simulink model "modelClampedBeam"  (R2024b)
settings: Solver=ode4  StartTime=0.0  StopTime=inf  FixedStep=settings.samplingTime_s  MaxStep=1e-2  RelTol=1e-5
PostLoadFcn:
  | , if any(exist('dsrtsu_mdlpostloadfcn', 'file') == [2, 3, 6]), try dsrtsu_mdlpostloadfcn('Execute', bdroot); catch fprintf('Error in PostLoadFcn (dsrtsu_mdlpostloadfcn) for model "%s":\n %s\n', bdroot, lasterr); end, end,
  | , if any(exist('dsrtsu_mdlpostloadfcn', 'file') ~= 0), dsrtsu_mdlpostloadfcn('Execute', bdroot); end,
undefined symbols (not defined in the file or in its folder): virtualBeam
Description:
  | Standard RTI1202 template.
  | Supported MATLAB version:  R2019b.
settings Model: Tag=RTI1202  DSRTSU_INTERNAL_RTI_VER=490  DSRTSU_INTERNAL_RTI_TYPE=rti1202  RTICANMMDATA=struct('GeneralSetupData',struct('modelroot','C:\UNI\Master\04_MA\05_Experiments','generalsettings',struct('filesettings',struct('destfolder',struct('Name','RTICANMM_FILES','Check',1),'buildfolder',struct('Name','.','Check',1),'AbsDestfolder',struct('Name','C:\UNI\Master\04_MA\05_Experiments\RTICANMM_FILES'),'AbsBuildfolder',struct('Name','C:\UNI\Master\04_MA\05_Experiments'))),'options',struct('addpaths',1,'rmpaths',1,'addtrcexclusion',true,'cannavigator',struct('checkmonitoring',0),'show_usrtrc',0,'use_usrtrc',0),'advanced',struct('options',ones(1,100)),'MPSetup',{{}},'RTI',struct('Type','RTI1202','Ver','7.13','Date','02-Nov-2019'),'modelname','PLL_autoStep_r2019b_rti','block','PLL_autoStep_r2019b_rti'))  DSRTSU_INTERNAL_RTIFPGA=80  Creator=patri  LastModifiedBy=phippold
settings SolverCC: AlgebraicLoopSolver=TrustRegion
settings DataIOCC: ReturnWorkspaceOutputs=off
settings OptimizationCC: BlockReduction=off  OptimizeBlockIOStorage=off  BufferReuse=off  GlobalBufferReuse=off  ExpressionFolding=off  LocalBlockOutputs=off
settings DebuggingCC: UnconnectedInputMsg=warning  UnconnectedOutputMsg=warning  UnconnectedLineMsg=warning  ArithmeticOperatorsInVariantConditions=warning
settings HardwareCC: TargetIntDivRoundTo=Zero  TargetEndianess=BigEndian  TargetHWDeviceType=Custom Processor->Custom
settings ModelReferenceCC: EnableRefExpFcnMdlSchedulingChecks=on
settings SFSimCC: SimUseLocalCustomCode=off  CustomCodeUndefinedFunction=UseInterfaceOnly
settings RTWCC: RTWUseLocalCustomCode=off  GPUComputeCapability=3.5  DLArmComputeVersion=19.05
settings CodeAppCC: StateflowObjectComments=on
settings ConfigComp: CovMetricSettings=dswe
settings SimscapeCC: SimscapeNormalizeSystem=off

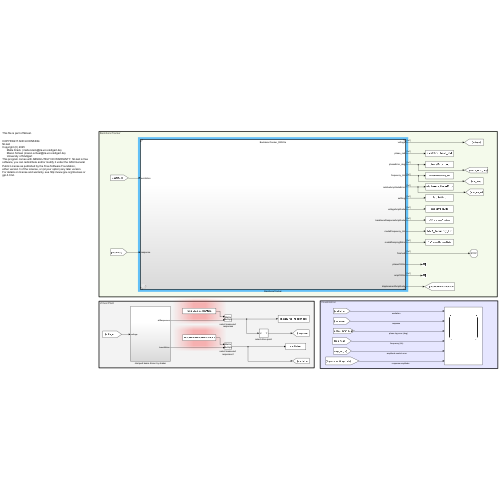
[thumbnail: Simulink's stored preview of the top-level diagram]
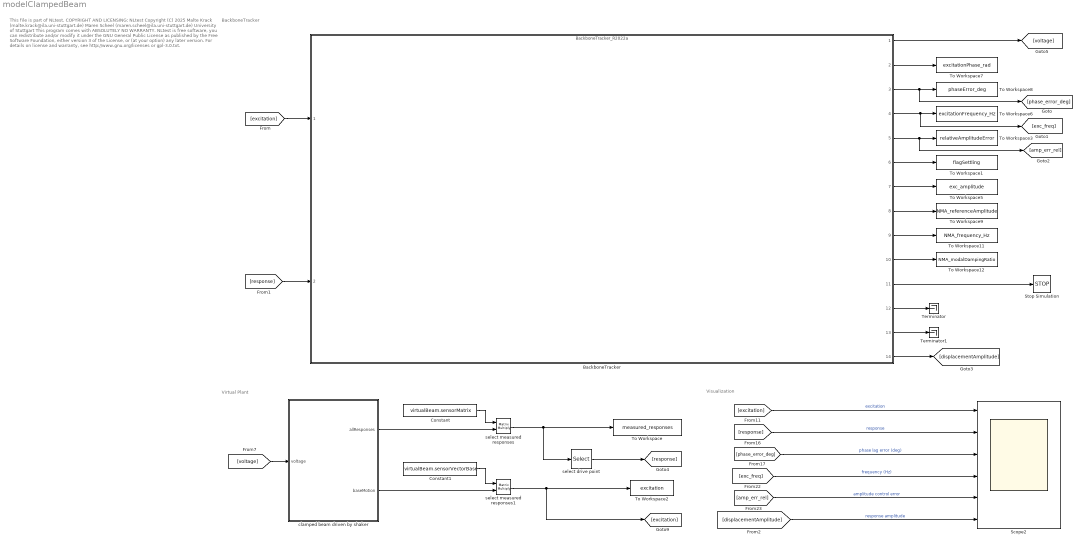
== system modelClampedBeam ==
  note: BackboneTracker
  note: Visualization
  note: Virtual Plant
  note: This file is part of NLtest.
      |
      | COPYRIGHT AND LICENSING:
      | NLtest
      | Copyright (C) 2025
      | Malte Krack (malte.krack@ila.uni-stuttgart.de)
      | Maren Scheel (maren.scheel@ila.uni-stuttgart.de)
      | University of Stuttgart
      | This program comes with ABSOLUTELY NO WARRANTY. NLtest is free software, you can redistribute and/or modify it under the GNU General Public License as published by the Free Software Foundation,
      | either version 3 of the License, or (at your option) any later version.
      | For details on license and warranty, see http://www.gnu.org/licenses or gpl-3.0.txt.
  BackboneTracker : ModelReference  ModelNameDialog=BackboneTracker_R2022a.slx  SimulationMode=Normal  ModelReferenceVersion=17.10
  Constant : Constant  Value=virtualBeam.sensorMatrix
  Constant1 : Constant  Value=virtualBeam.sensorVectorBase  VectorParams1D=off
  Scope2 : Scope  NumInputPorts=6
  Stop Simulation : Stop
  Terminator : Terminator
  Terminator1 : Terminator
  To Workspace : ToWorkspace  VariableName=measured_responses  SaveFormat=Structure With Time  SampleTime=-1
  To Workspace1 : ToWorkspace  VariableName=flagSettling  SaveFormat=Structure With Time  SampleTime=-1
  To Workspace11 : ToWorkspace  VariableName=NMA_frequency_Hz  SaveFormat=Structure With Time  SampleTime=-1
  To Workspace12 : ToWorkspace  VariableName=NMA_modalDampingRatio  SaveFormat=Structure With Time  SampleTime=-1
  To Workspace2 : ToWorkspace  VariableName=excitation  SaveFormat=Structure With Time  SampleTime=-1
  To Workspace3 : ToWorkspace  VariableName=relativeAmplitudeError  SaveFormat=Structure With Time  SampleTime=-1
  To Workspace5 : ToWorkspace  VariableName=exc_amplitude  SaveFormat=Structure With Time  SampleTime=-1
  To Workspace6 : ToWorkspace  VariableName=excitationFrequency_Hz  SaveFormat=Structure With Time  SampleTime=-1
  To Workspace7 : ToWorkspace  VariableName=excitationPhase_rad  SaveFormat=Structure With Time  SampleTime=-1
  To Workspace8 : ToWorkspace  VariableName=phaseError_deg  SaveFormat=Structure With Time  SampleTime=-1
  To Workspace9 : ToWorkspace  VariableName=NMA_referenceAmplitude  SaveFormat=Structure With Time  SampleTime=-1
  clamped beam driven by shaker : Subsystem
  select drive point : Selector  IndexOptions=Index vector (dialog)  Indices=settings.indexSensorControl  OutputSizes=1
  select measured responses : Product  Multiplication=Matrix(*)
  select measured responses1 : Product  Multiplication=Matrix(*)
  wires:
  select measured responses/1 -> To Workspace/1, select drive point/1
  [voltage] -> clamped beam driven by shaker/1(voltage)
  [excitation] -> Scope2/1  "excitation"
  [response] -> Scope2/2  "response"
  [phase_error_deg] -> Scope2/3  "phase lag error (deg)"
  [exc_freq] -> Scope2/4  "frequency (Hz)"
  [amp_err_rel] -> Scope2/5  "amplitude control error"
  [displacementAmplitude] -> Scope2/6  "response amplitude"
  select drive point/1 -> [response]
  BackboneTracker/2 -> To Workspace7/1
  BackboneTracker/3 -> [phase_error_deg], To Workspace8/1
  BackboneTracker/5 -> [amp_err_rel], To Workspace3/1
  BackboneTracker/4 -> [exc_freq], To Workspace6/1
  BackboneTracker/6 -> To Workspace1/1
  BackboneTracker/7 -> To Workspace5/1
  BackboneTracker/10 -> To Workspace12/1
  BackboneTracker/9 -> To Workspace11/1
  BackboneTracker/8 -> To Workspace9/1
  BackboneTracker/11 -> Stop Simulation/1
  BackboneTracker/12 -> Terminator/1
  BackboneTracker/13 -> Terminator1/1
  BackboneTracker/1 -> [voltage]
  [excitation] -> BackboneTracker/1
  [response] -> BackboneTracker/2
  clamped beam driven by shaker/1(allResponses) -> select measured responses/2
  Constant/1 -> select measured responses/1
  BackboneTracker/14 -> [displacementAmplitude]
  select measured responses1/1 -> To Workspace2/1, [excitation]
  Constant1/1 -> select measured responses1/1
  clamped beam driven by shaker/2(baseMotion) -> select measured responses1/2

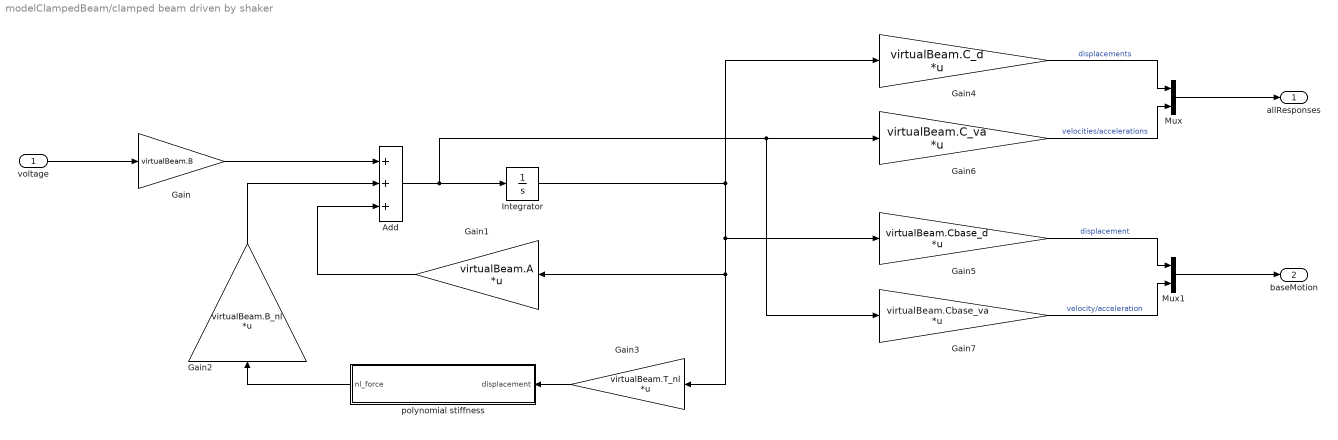
== system modelClampedBeam/clamped beam driven by shaker ==
  voltage : Inport
  Add : Sum  Inputs=+++
  Gain : Gain  Gain=virtualBeam.B
  Gain1 : Gain  Gain=virtualBeam.A  Multiplication=Matrix(K*u) (u vector)
  Gain2 : Gain  Gain=virtualBeam.B_nl  Multiplication=Matrix(K*u) (u vector)
  Gain3 : Gain  Gain=virtualBeam.T_nl  Multiplication=Matrix(K*u)
  Gain4 : Gain  Gain=virtualBeam.C_d  Multiplication=Matrix(K*u) (u vector)
  Gain5 : Gain  Gain=virtualBeam.Cbase_d  Multiplication=Matrix(K*u) (u vector)
  Gain6 : Gain  Gain=virtualBeam.C_va  Multiplication=Matrix(K*u) (u vector)
  Gain7 : Gain  Gain=virtualBeam.Cbase_va  Multiplication=Matrix(K*u) (u vector)
  Integrator : Integrator
  Mux : Mux  Inputs=2
  Mux1 : Mux  Inputs=2
  polynomial stiffness : Subsystem
  allResponses : Outport
  baseMotion : Outport  Port=2
  wires:
  voltage/1 -> Gain/1
  Gain/1 -> Add/1
  Add/1 -> Integrator/1, Gain7/1, Gain6/1
  Gain1/1 -> Add/3
  Gain2/1 -> Add/2
  polynomial stiffness/1(nl_force) -> Gain2/1
  Gain3/1 -> polynomial stiffness/1(displacement)
  Integrator/1 -> Gain5/1, Gain1/1, Gain3/1, Gain4/1
  Gain4/1 -> Mux/1  "displacements"
  Gain6/1 -> Mux/2  "velocities/accelerations"
  Mux/1 -> allResponses/1
  Gain7/1 -> Mux1/2  "velocity/acceleration"
  Gain5/1 -> Mux1/1  "displacement"
  Mux1/1 -> baseMotion/1

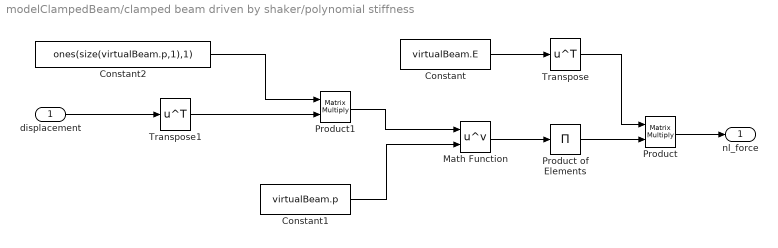
== system modelClampedBeam/clamped beam driven by shaker/polynomial stiffness ==
  displacement : Inport
  Constant : Constant  Value=virtualBeam.E
  Constant1 : Constant  Value=virtualBeam.p
  Constant2 : Constant  Value=ones(size(virtualBeam.p,1),1)
  Math Function : Math  Operator=pow
  Product : Product  Multiplication=Matrix(*)
  Product of Elements : Product  Inputs=*  CollapseMode=Specified dimension  CollapseDim=2
  Product1 : Product  Multiplication=Matrix(*)
  Transpose : Math  Operator=transpose
  Transpose1 : Math  Operator=transpose
  nl_force : Outport
  wires:
  Product of Elements/1 -> Product/2
  Product/1 -> nl_force/1
  Constant/1 -> Transpose/1
  Transpose/1 -> Product/1
  Product1/1 -> Math Function/1
  Math Function/1 -> Product of Elements/1
  Constant1/1 -> Math Function/2
  Constant2/1 -> Product1/1
  displacement/1 -> Transpose1/1
  Transpose1/1 -> Product1/2
